simulink model "YMBOX_Control_Core"  (R2024b)
settings: Solver=FixedStepDiscrete  StartTime=0.0  StopTime=3  RelTol=1e-3
PreLoadFcn:
  | run(fullfile(fileparts(get_param(bdroot,'FileName')), 'YMBOX_Deluxe_init.m'));
InitFcn:
  | YMBOX_InitializeModel('core',bdroot);
model workspace (MAT data in the model file):
  KuMDAS_ObserverBuildVariant = Simulink.Parameter
  KuMDAS_ObserverBuildVariant.Value = 1
  KuMDAS_ObserverBuildVariant.Complexity = 'real'
  KuMDAS_ObserverBuildVariant.Dimensions = [1 1]
  KuMDAS_ObserverBuildVariant.Description = 'Product observer build Variant: 0=sensored-only, 1=SMO sensorless'
  KuMDAS_ObserverBuildVariant.DataType = 'uint8'
undefined symbols (not defined in the file or in its folder): CeMDSM_DrvModeIfStart_enum, CeMDSM_DrvModeSpdSens_enum, CeMDSM_DrvModeSpdSmo_enum, CeMDSM_DrvModeTrq_enum, Cf_CONTROL_TASK_TIME_S, KbMDAS_SmoDeadTimeCompEnable_flg, KbMDSA_ActiveInverterCompEnable_flg, KbMDSA_UnifiedVoltageLimitEnable_flg, KbMDSP_DCBusVoltReportFilterEnable_flg, KbMDTM_DAxisPriorityInFW_flg, KbMDTM_FieldWeakeningEnable_flg, KbMDTM_FinalIqAntiWindupEnable_flg, KbMDTM_SensorlessFieldWeakeningEnable_flg, KbMDTM_TorquePriorityBelowBase_flg, KbMDTM_UnifiedConstraintEnable_flg, KfMDAS_ControlCountToElecRad_NULL, KfMDAS_IfAccel_rpms, KfMDAS_IfAlignTime_s, KfMDAS_IfBlendTime_s, KfMDAS_IfSwitchSpd_rpm, KfMDAS_NativeCountToMechRad_NULL, KfMDAS_ObserverExitRatio_NULL, KfMDAS_SlsCtrlPeriod_s, KfMDAS_SlsEAngleInit_rad, KfMDAS_SlsElecSpdMax_rads, KfMDAS_SlsElecSpdMin_rads, KfMDAS_SlsTwoPi_rad, KfMDAS_SmoAngleOffset_rad, KfMDAS_SmoCurrentZohCoefA_NULL, KfMDAS_SmoCurrentZohCoefB_AperV, KfMDAS_SmoDeadTimeCurrentBoundary_A, KfMDAS_SmoDeadTimeDuty_NULL, KfMDAS_SmoDeadTimePolarity_NULL, KfMDAS_SmoDeviceDrop_V, KfMDAS_SmoEmfLpfCoefA_NULL, KfMDAS_SmoEmfLpfCoefB_NULL, KfMDAS_SmoEmfLpfInvPole_s, KfMDAS_SmoErrBoundaryMax_A, KfMDAS_SmoErrBoundarySpan_A, KfMDAS_SmoGainSchedAlpha_NULL, KfMDAS_SmoGainSchedAngleComp_rad, KfMDAS_SmoGainSchedEmfLow_V, KfMDAS_SmoGainSchedInvSpan_PerV, KfMDAS_SmoLdMinusLq_H, KfMDAS_SmoPllKiTs_NULL, KfMDAS_SmoPllKp_NULL, KfMDAS_SmoPllMinEmf_V, KfMDAS_SmoPllSpeedLpfAlpha_NULL, KfMDAS_SmoSlideGainMin_V, KfMDAS_SmoSlideGainSpan_V, KfMDAS_SmoSwitchSpd_rpm, KfMDAS_SmoTotalDelay_s, KfMDCC_DqSoftwareOverCurrentThreshold_A, KfMDCC_PiKcTsId_NULL, KfMDCC_PiKcTsIq_NULL, KfMDCC_PiKiTsId_NULL, KfMDCC_PiKiTsIq_NULL, KfMDCC_PiKpValueId_NULL, KfMDCC_PiKpValueIq_NULL, KfMDCC_PwmFreq_Hz ... (+84)
libraries: YMBOX_SharedMath_Lib x11, spsabctoAlphaBetaZeroLib x1
(part 1 of 8)
settings Model: Creator=ASUS  LastModifiedBy=ASUS
settings SolverCC: AlgebraicLoopSolver=TrustRegion  AutoInsertRateTranBlk=on
settings DataIOCC: LimitDataPoints=on  SaveFormat=StructureWithTime  SignalLoggingSaveFormat=ModelDataLogs  SaveOutput=off  SaveTime=off  ReturnWorkspaceOutputs=off
settings OptimizationCC: BlockReduction=off  ConditionallyExecuteInputs=off  DefaultParameterBehavior=Inlined  DefaultUnderspecifiedDataType=single  EnhancedBackFolding=on  PassReuseOutputArgsAs=Individual arguments  ExpressionDepthLimit=2147483647  InitFltsAndDblsToZero=on  EfficientFloat2IntCast=on  EfficientMapNaN2IntZero=off  OptimizeBlockOrder=speed  DifferentSizesBufferReuse=on  OptimizationCustomize=off  EfficientTunableParamExpr=on
settings DebuggingCC: ConsistencyChecking=warning  SignalInfNanChecking=error  SignalRangeChecking=error  SaveWithParameterizedLinksMsg=none  CheckSSInitialOutputMsg=off  UnderspecifiedInitializationDetection=Classic  MergeDetectMultiDrivingBlocksExec=none  TimeAdjustmentMsg=warning  MaxConsecutiveZCsMsg=warning  SolverPrmCheckMsg=warning  InheritedTsInSrcMsg=none  CheckMatrixSingularityMsg=error  ParameterOverflowMsg=warning  ParameterUnderflowMsg=error  ParameterPrecisionLossMsg=none  FixptConstUnderflowMsg=warning  FixptConstOverflowMsg=warning  FixptConstPrecisionLossMsg=warning  VectorMatrixConversionMsg=warning  FcnCallInpInsideContextMsg=warning  UnconnectedInputMsg=warning  UnconnectedOutputMsg=warning  UnconnectedLineMsg=warning  UniqueDataStoreMsg=warning  AllowSymbolicDim=off  StateNameClashWarn=warning  SFUnexpectedBacktrackingDiag=warning  SFNoUnconditionalDefaultTransitionDiag=warning  SFExecutionAtInitializationDiag=none  ArithmeticOperatorsInVariantConditions=warning
settings HardwareCC: ProdBitPerChar=16  ProdBitPerInt=16  ProdBitPerPointer=32  ProdBitPerSizeT=32  ProdBitPerPtrDiffT=32  ProdLargestAtomicInteger=Integer  ProdLargestAtomicFloat=None  ProdWordSize=16  ProdHWDeviceType=Texas Instruments->C2000  TargetIntDivRoundTo=Zero  TargetEndianess=LittleEndian  TargetHWDeviceType=Infineon->TriCore  ProdEqTarget=off
settings ModelReferenceCC: EnableRefExpFcnMdlSchedulingChecks=on  ModelReferenceNumInstancesAllowed=Single  PropagateSignalLabelsOutOfModel=off
settings SFSimCC: SimUseLocalCustomCode=off  MATLABDynamicMemAlloc=off  CustomCodeUndefinedFunction=UseInterfaceOnly
settings SFSimCC: SimCustomSourceCode=|
  | void Pwm_SetOutputToIdle_Now(void){};
  | void InverterDisable(void){};
  | void Pwm_Write(void){};
  | void InverterEnable(void){};
  | void vPwm_MDCC_UdUqCalc1_PI_Self_initialize(void){};
  | void SpeedLoopMode_initialize(void){};
settings SFSimCC: SimCustomHeaderCode=|
  | void Pwm_SetOutputToIdle_Now(void);
  | void InverterDisable(void);
  | void Pwm_Write(void);
  | void InverterEnable(void);
  | void vPwm_MDCC_UdUqCalc1_PI_Self_initialize(void);
  | void SpeedLoopMode_initialize(void);
  | #include "mdsa_sincos_f32.h"
  | #include "ymbox_atan_f32.h"
  | #include "ymbox_sqrt_f32.h"
  | #include "ymbox_scalar_math_f32.h"
settings SFSimCC: SimCustomInitializer=|
  | MDSA_SinCos_Init();
  | YMBOX_Atan_Init();
  | YMBOX_Sqrt_Init();
settings SFSimCC: SimUserSources=|
  | Platform/SinCos/mdsa_sincos_generic.c
  | Platform/Atan/ymbox_atan_generic.c
  | Platform/Sqrt/ymbox_sqrt_generic.c
  | Platform/SharedMath/ymbox_scalar_math_f32.c
settings SFSimCC: SimUserIncludeDirs=|
  | Platform/SinCos
  | Platform/Atan
  | Platform/Sqrt
  | Platform/SharedMath
settings RTWCC: Description=Embedded Coder  SystemTargetFile=ert.tlc  TLCOptions=-p0  GenCodeOnly=on  TemplateMakefile=ert_default_tmf  GenerateReport=on  RTWUseLocalCustomCode=off  IncludeHyperlinkInReport=on  GPUComputeCapability=3.5
settings RTWCC: CustomHeaderCode=|
  | extern void Pwm_SetOutputToIdle_Now(void);
  | extern void InverterDisable(void);
  | extern void Pwm_Write(void);
  | extern void InverterEnable(void);
  | void vPwm_MDCC_UdUqCalc1_PI_Self_initialize(void);
  | void SpeedLoopMode_initialize(void);
  | #include "mdsa_sincos_f32.h"
  | #include "ymbox_atan_f32.h"
  | #include "ymbox_sqrt_f32.h"
  | #include "ymbox_scalar_math_f32.h"
settings RTWCC: CustomInclude=|
  | Platform/SinCos
  | Platform/Atan
  | Platform/Sqrt
  | Platform/SharedMath
settings CodeAppCC: GenerateComments=off  IgnoreCustomStorageClasses=off  MaxIdLength=100  OperatorAnnotations=on  SFDataObjDesc=on  CustomSymbolStrGlobalVar=rt$N$M  CustomSymbolStrType=$N$M  CustomSymbolStrFcn=$N$M$F  CustomSymbolStrMacro=$N$M  CustomCommentsFcn=comments_mptfun.m  DefineNamingRule=UpperCase  SimulinkBlockComments=off  InternalIdentifier=Classic
settings ERTTargetCC: TargetLangStandard=C99 (ISO)  CodeReplacementLibrary=YMBOX single math  GenerateSampleERTMain=on  ERTCustomFileTemplate=example_file_process.tlc
settings ConfigComp: CovMetricSettings=dw  CovSaveCumulativeToWorkspaceVar=on  CovSaveSingleToWorkspaceVar=on  CovExternalEMLEnable=off

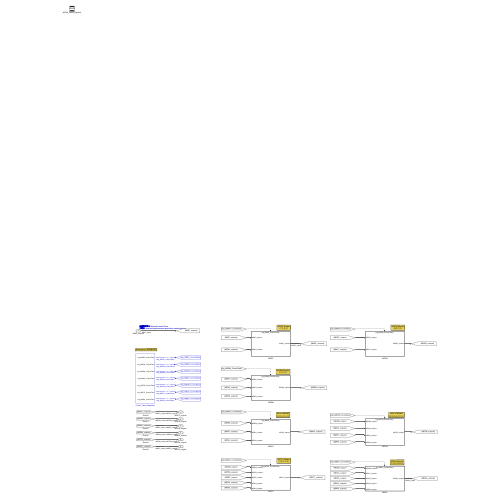
[thumbnail: Simulink's stored preview of the top-level diagram]
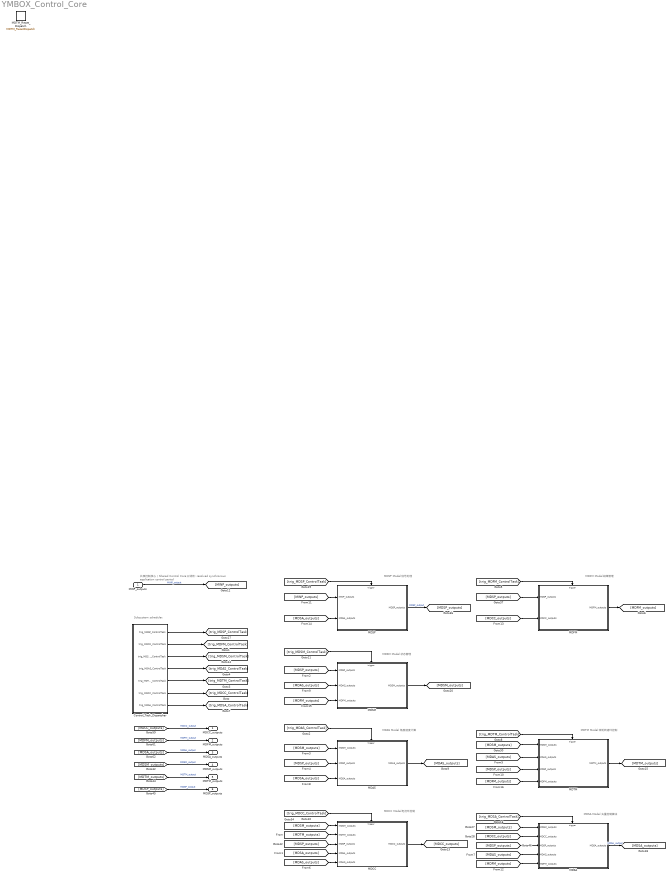
== system YMBOX_Control_Core ==
  note: Subsystem scheduler.
  note: MDFM Model
      | 故障管理
  note: MDCC Model
      | 电流环控制
  note: MDSA Model
      | 矢量控制算法
  note: MDTM Model
      | 转矩转速环控制
  note: MDSM Model
      | 状态管理
  note: MDAS Model
      | 角度速度计算
  note: 共享控制核心 / Shared Control Core
      | 父调用: resolved synchronous application control period
  note: MDSP Model
      | 信号处理
  MINP_outputs : Inport  OutDataTypeStr=Bus: MINP_output
  Control_Task_Dispatcher : Subsystem
  MDAS : Subsystem  TreatAsAtomicUnit=on  RTWFileName=AUXV_control
      settings: RTWSystemCode=Nonreusable function  RTWFileNameOpts=Use subsystem name
  MDCC : Subsystem  TreatAsAtomicUnit=on  RTWFileName=AUXV_control
      settings: RTWSystemCode=Nonreusable function  RTWFileNameOpts=Use subsystem name
  MDFM : Subsystem  TreatAsAtomicUnit=on  RTWFileName=AUXV_control
      settings: RTWSystemCode=Nonreusable function  RTWFileNameOpts=Use subsystem name
  MDSA : Subsystem  TreatAsAtomicUnit=on  RTWFileName=AUXV_control
      settings: RTWSystemCode=Nonreusable function  RTWFileNameOpts=Use subsystem name
  MDSM : Subsystem  TreatAsAtomicUnit=on  RTWFileName=AUXV_control
      settings: RTWSystemCode=Nonreusable function  RTWFileNameOpts=Use subsystem name
  MDSP : Subsystem
  MDTM : Subsystem  TreatAsAtomicUnit=on  RTWFileName=AUXV_control
      settings: RTWSystemCode=Nonreusable function  RTWFileNameOpts=Use subsystem name
  MDTM_Reset_Dispatch : DataStoreMemory  Description=MDSM writes the current fast-tick reset request before Scheduler reads it. Read only after trig_MDSM_ControlTask returns.  DataStoreName=MDTM_ResetDispatch  InitialValue=false  ShowAdditionalParam=off  OutDataTypeStr=boolean
  MDCC_outputs : Outport  OutDataTypeStr=Bus: MDCC_output
  MDFM_outputs : Outport  Port=2  OutDataTypeStr=Bus: MDFM_output
  MDSA_outputs : Outport  Port=3  OutDataTypeStr=Bus: MDSA_output
  MDSM_outputs : Outport  Port=4  OutDataTypeStr=Bus: MDSM_output
  MDTM_outputs : Outport  Port=5  OutDataTypeStr=Bus: MDTM_output
  MDSP_outputs : Outport  Port=6  OutDataTypeStr=Bus: MDSP_output
  wires:
  [MDFM_outputs] -> MDFM_outputs/1  "MDFM_output"
  [MDCC_outputs] -> MDCC_outputs/1  "MDCC_output"
  Control_Task_Dispatcher/5(trig_MDTM_ControlTask) -> [trig_MDTM_ControlTask]
  Control_Task_Dispatcher/7(trig_MDSA_ControlTask) -> [trig_MDSA_ControlTask]
  Control_Task_Dispatcher/6(trig_MDCC_ControlTask) -> [trig_MDCC_ControlTask]
  Control_Task_Dispatcher/2(trig_MDFM_ControlTask) -> [trig_MDFM_ControlTask]
  [MDSA_outputs] -> MDSA_outputs/1  "MDSA_output"
  Control_Task_Dispatcher/3(trig_MDSM_ControlTask) -> [trig_MDSM_ControlTask]
  [MDTM_outputs] -> MDTM_outputs/1  "MDTM_output"
  [MDSM_outputs] -> MDSM_outputs/1  "MDSM_output"
  [trig_MDFM_ControlTask] -> MDFM/Trigger
  MDFM/1(MDFM_outputs) -> [MDFM_outputs]
  [trig_MDCC_ControlTask] -> MDCC/Trigger
  MDCC/1(MDCC_outputs) -> [MDCC_outputs]
  [trig_MDSA_ControlTask] -> MDSA/Trigger
  MDSA/1(MDSA_outputs) -> [MDSA_outputs]  "MDSA_output"
  [trig_MDTM_ControlTask] -> MDTM/Trigger
  MDTM/1(MDTM_outputs) -> [MDTM_outputs]
  [trig_MDSM_ControlTask] -> MDSM/Trigger
  MDSM/1(MDSM_outputs) -> [MDSM_outputs]
  [MDSM_outputs] -> MDSA/1(MDSM_outputs)
  [MDCC_outputs] -> MDSA/2(MDCC_outputs)
  [MDSM_outputs] -> MDTM/1(MDSM_outputs)
  [MDSM_outputs] -> MDCC/1(MDSM_outputs)
  [MDTM_outputs] -> MDCC/2(MDTM_outputs)
  [MDSP_outputs] -> MDFM/1(MDSP_outputs)
  [MDSP_outputs] -> MDCC/3(MDSP_outputs)
  [MDSP_outputs] -> MDSA/3(MDSP_outputs)
  [MDSP_outputs] -> MDSP_outputs/1  "MDSP_output"
  [MDSP_outputs] -> MDSM/1(MDSP_outputs)
  [MDSA_outputs] -> MDCC/4(MDSA_outputs)
  Control_Task_Dispatcher/4(trig_MDAS_ControlTask) -> [trig_MDAS_ControlTask]
  [trig_MDAS_ControlTask] -> MDAS/Trigger
  [MDSM_outputs] -> MDAS/1(MDSM_outputs)
  [MDSP_outputs] -> MDAS/2(MDSP_outputs)
  MDAS/1(MDAS_outputs) -> [MDAS_outputs]
  [MDAS_outputs] -> MDTM/2(MDAS_outputs)
  [MDAS_outputs] -> MDCC/5(MDAS_outputs)
  [MDAS_outputs] -> MDSA/4(MDAS_outputs)
  [MDSA_outputs] -> MDAS/3(MDSA_outputs)
  [MDAS_outputs] -> MDSM/2(MDAS_outputs)
  [MDSP_outputs] -> MDTM/3(MDSP_outputs)
  MDSP/1(MDSP_outputs) -> [MDSP_outputs]  "MDSP_output"
  MINP_outputs/1 -> [MINP_outputs]  "MINP_output"
  [MINP_outputs] -> MDSP/1(MINP_outputs)
  [trig_MDSP_ControlTask] -> MDSP/Trigger
  Control_Task_Dispatcher/1(trig_MDSP_ControlTask) -> [trig_MDSP_ControlTask]
  [MDSA_outputs] -> MDSP/2(MDSA_outputs)
  [MDFM_outputs] -> MDSM/3(MDFM_outputs)
  [MDFM_outputs] -> MDTM/4(MDFM_outputs)
  [MDFM_outputs] -> MDSA/5(MDFM_outputs)
  [MDCC_outputs] -> MDFM/2(MDCC_outputs)

== system YMBOX_Control_Core/Control_Task_Dispatcher ==
  note: Scheduler to trigger the main application
      | sub-systems.
  Scheduler : Stateflow chart  TreatAsAtomicUnit=on
      settings: PortSchema="{\"entries\":[{\"content\":{\"sides\":[{\"content\":{},\"type\":\"ConnectorPlacement.EquallySpacedRectSide\",\"uuid\":\"ed742335-5841-4393-a6a4-c33eaa575858\"},{\"content\":{\"connectorIds\":[\"Out7\",\"Out1\",\"Out2\",\"Out3\",\"Out4\",\"Out5\",\"Out6\"],\"side\":\"RIGHT\"},\"type\":\"ConnectorPlacement.EquallySpacedRectSide\",\"uuid\":\"a5f78643-cf3a-43ed-917c-1379891acf9e\"},{\"content\":{\"side\":\"TOP\"},\"type\":\"ConnectorPlacement.EquallySpacedRectSide\",\"uuid\":\"5ceff9a0-c2d2-40e1-aa51-0f4c65c30636\"}]},\"type\":\"ConnectorPlacement.EquallySpacedConnector\",\"uuid\":\"5d18fd33-d652-411a-b3bb-ce8a67e81c97\"}],\"packageUris\":[\"http://schema.mathworks.com/mf0/Connector/R2020b\"],\"version\":\"1.0\"}"
  trig_MDSP_ControlTask : Outport
  trig_MDFM_ControlTask : Outport  Port=2
  trig_MDSM_ControlTask : Outport  Port=3
  trig_MDAS_ControlTask : Outport  Port=4
  trig_MDTM_ControlTask : Outport  Port=5
  trig_MDCC_ControlTask : Outport  Port=6
  trig_MDSA_ControlTask : Outport  Port=7
  wires:
  Scheduler/1(trig_MDFM_ControlTask()) -> trig_MDFM_ControlTask/1
  Scheduler/2(trig_MDSM_ControlTask()) -> trig_MDSM_ControlTask/1
  Scheduler/3(trig_MDAS_ControlTask()) -> trig_MDAS_ControlTask/1
  Scheduler/4(trig_MDTM_ControlTask()) -> trig_MDTM_ControlTask/1
  Scheduler/5(trig_MDCC_ControlTask()) -> trig_MDCC_ControlTask/1
  Scheduler/6(trig_MDSA_ControlTask()) -> trig_MDSA_ControlTask/1
  Scheduler/7(trig_MDSP_ControlTask()) -> trig_MDSP_ControlTask/1

== system YMBOX_Control_Core/MDAS ==
  MDSM_outputs : Inport
  MDSP_outputs : Inport  Port=2
  MDSA_outputs : Inport  Port=3
  trig_MDAS_ControlTask : TriggerPort  TriggerType=function-call  VariantControl=(inherit)
  Bus Creator : BusCreator  Inputs=12  OutDataTypeStr=Bus: MDAS_output
  Bus Selector : BusSelector  OutputSignals=VeMDSM_DrvModeCmd_enum,VeMDSM_DrvModeReq_enum,VfMDSM_TrgtSpd_rpm
  Bus Selector1 : BusSelector  OutputSignals=Resolver_Output.VuMDSP_MotMechAngleRaw_NULL
  IF_Startup_Internal : Subsystem  Variant=on
      settings: AttributesFormatString=PRODUCT BUILD VARIANT\n0 SENSORED | 1 SMO
  MDAS_DriveModeRoute_Variant : Subsystem  Variant=on
      settings: AttributesFormatString=PRODUCT BUILD VARIANT\n0 SENSORED | 1 SMO
  MechSpd_To_ElecSpd : Gain  Gain=single(KuMDMP_Pole_Pair_Number_NULL)  OutDataTypeStr=single
  Position_Feedback_Status : Stateflow chart  TreatAsAtomicUnit=on
  Position_NativeCountToMechRad : Constant  Value=KfMDAS_NativeCountToMechRad_NULL
  Position_TwoPiRad : Constant  Value=KfMDAS_SlsTwoPi_rad
  Sensorless_FluxMRAS : Subsystem  Variant=on  VariantControl=Sensorless_FluxMRAS
      settings: AttributesFormatString=PRODUCT BUILD VARIANT\n0 SENSORED | 1 SMO
  MDAS_outputs : Outport  OutDataTypeStr=Bus: MDAS_output
  wires:
  MDSM_outputs/1 -> Bus Selector/1, Sensorless_FluxMRAS/3(MDSM_outputs)
  [MDAS_SMO_ELEC_ANGLE_RAD_ROUTE] -> MDAS_DriveModeRoute_Variant/8(VfMDAS_SmoAlignedElecAngle_rad)
  MDSA_outputs/1 -> Sensorless_FluxMRAS/2(MDSA_outputs)
  [MDAS_RAW_ANGLE_ROUTE] -> Position_Feedback_Status/2(rawMechCount), MDAS_DriveModeRoute_Variant/2(<VuMDSP_MotMechAngleRaw_NULL>)
  [MDAS_SMO_ABS_ROUTE] -> MDAS_DriveModeRoute_Variant/5(VfMDAS_SmoMechSpdAbs_rads)
  MDSP_outputs/1 -> Bus Selector1/1, Sensorless_FluxMRAS/1(MDSP_outputs)
  [MDAS_IF_ABS_ROUTE] -> MDAS_DriveModeRoute_Variant/3(VfMDAS_IfMechSpdAbs_rads)
  [MDAS_MODE_CMD_ROUTE] -> MDAS_DriveModeRoute_Variant/1(<VeMDSM_DrvModeCmd_enum>), Position_Feedback_Status/1(modeCmd)
  [MDAS_IF_ELEC_ANGLE_RAD_ROUTE] -> MDAS_DriveModeRoute_Variant/7(VfMDAS_IfElecAngle_rad)
  [MDAS_IF_SPD_ROUTE] -> MDAS_DriveModeRoute_Variant/4(VfMDAS_IfMechSpd_rads)
  [MDAS_READY_BUS] -> Bus Creator/4, Position_Feedback_Status/5(smoReady)
  [MDAS_SMO_SPD_ROUTE] -> MDAS_DriveModeRoute_Variant/6(VfMDAS_SmoMechSpd_rads)
  Bus Selector/1 -> [MDAS_MODE_CMD_ROUTE], IF_Startup_Internal/1(VeMDAS_DrvModeCmd_enum)  "<VeMDSM_DrvModeCmd_enum>"
  Position_Feedback_Status/1(mechAngleRad) -> Bus Creator/7  "VfMDAS_MotMechAngle_rad"
  Bus Selector/2 -> IF_Startup_Internal/2(VeMDAS_DrvModeReq_enum)  "<VeMDSM_DrvModeReq_enum>"
  Bus Selector1/1 -> [MDAS_RAW_ANGLE_ROUTE]  "<VuMDSP_MotMechAngleRaw_NULL>"
  Bus Selector/3 -> IF_Startup_Internal/3(VfMDAS_TargetSpd_rpm)  "<VfMDSM_TrgtSpd_rpm>"
  Sensorless_FluxMRAS/1(VfMDAS_SmoElecAngle_rad) -> IF_Startup_Internal/4(VfMDAS_SmoElecAngle_rad)
  Sensorless_FluxMRAS/2(VfMDAS_SmoElecSpd_rads) -> IF_Startup_Internal/5(VfMDAS_SmoElecSpd_rads)
  IF_Startup_Internal/9(VfMDAS_HandoverElecAngleDelta_rad) -> [MDAS_HANDOVER_ELEC_ANGLE_DELTA_RAD]  "VfMDAS_HandoverElecAngleDelta_rad"
  Sensorless_FluxMRAS/3(VfMDAS_SmoEmfMag_V) -> IF_Startup_Internal/6(VfMDAS_SmoEmfMag_V)
  IF_Startup_Internal/4(VfMDAS_SmoMechSpd_rads) -> [MDAS_SMO_SPD_ROUTE]  "VfMDAS_SmoMechSpd_rads"
  IF_Startup_Internal/3(VfMDAS_IfElecAngle_rad) -> [MDAS_IF_ELEC_ANGLE_RAD_ROUTE]  "VfMDAS_IfElecAngle_rad"
  IF_Startup_Internal/2(VfMDAS_IfMechSpdAbs_rads) -> [MDAS_IF_ABS_ROUTE]  "VfMDAS_IfMechSpdAbs_rads"
  IF_Startup_Internal/1(VfMDAS_IfMechSpd_rads) -> [MDAS_IF_SPD_ROUTE]  "VfMDAS_IfMechSpd_rads"
  Sensorless_FluxMRAS/4(VfMDAS_SmoPllPhaseErr_NULL) -> IF_Startup_Internal/7(VfMDAS_SmoPllPhaseErr_NULL)
  MDAS_DriveModeRoute_Variant/3(VfMDAS_SelectedElecAngle_rad) -> Position_Feedback_Status/3(selectedElecAngleRad)  "VfMDAS_SelectedElecAngle_rad"
  MDAS_DriveModeRoute_Variant/2(VfMDAS_MotMechSpdFiltered_rads) -> Position_Feedback_Status/4(selectedMechSpdRads), Bus Creator/1, MechSpd_To_ElecSpd/1  "VfMDAS_MotMechSpdFiltered_rads"
  MDAS_DriveModeRoute_Variant/1(VfMDAS_MotMechSpdFilteredAbs_rads) -> Bus Creator/2  "VfMDAS_MotMechSpdFilteredAbs_rads"
  Position_NativeCountToMechRad/1 -> Position_Feedback_Status/6(nativeToMech)
  Position_TwoPiRad/1 -> Position_Feedback_Status/7(twoPiRad)
  IF_Startup_Internal/8(VfMDAS_HandoverBlend_NULL) -> [MDAS_BLEND_BUS]  "VfMDAS_HandoverBlend_NULL"
  IF_Startup_Internal/7(VfMDAS_SmoAlignedElecAngle_rad) -> [MDAS_SMO_ELEC_ANGLE_RAD_ROUTE]  "VfMDAS_SmoAlignedElecAngle_rad"
  IF_Startup_Internal/6(VbMDAS_SmoReady_flg) -> [MDAS_READY_BUS]  "VbMDAS_SmoReady_flg"
  IF_Startup_Internal/5(VfMDAS_SmoMechSpdAbs_rads) -> [MDAS_SMO_ABS_ROUTE]  "VfMDAS_SmoMechSpdAbs_rads"
  MechSpd_To_ElecSpd/1 -> Bus Creator/3  "VfMDAS_MotElecSpd_rads"
  [MDAS_BLEND_BUS] -> Bus Creator/5
  [MDAS_HANDOVER_ELEC_ANGLE_DELTA_RAD] -> Bus Creator/6
  Position_Feedback_Status/2(elecAngleRad) -> Bus Creator/8  "VfMDAS_MotElecAngle_rad"
  Position_Feedback_Status/3(angleValid) -> Bus Creator/9  "VbMDAS_PositionAngleValid_flg"
  Position_Feedback_Status/4(speedValid) -> Bus Creator/10  "VbMDAS_PositionSpeedValid_flg"
  Position_Feedback_Status/5(quality) -> Bus Creator/11  "VfMDAS_PositionQuality_NULL"
  Bus Creator/1 -> MDAS_outputs/1
  Position_Feedback_Status/6(direction) -> Bus Creator/12  "VeMDAS_PositionDirection_enum"

== system YMBOX_Control_Core/MDCC ==
  MDSM_outputs : Inport
  MDTM_outputs : Inport  Port=2
  MDSP_outputs : Inport  Port=3
  MDSA_outputs : Inport  Port=4
  MDAS_outputs : Inport  Port=5
  trig_MDCC_ControlTask : TriggerPort  TriggerType=function-call  VariantControl=(inherit)
  Bus Creator : BusCreator  Inputs=7
  Bus Selector1 : BusSelector  OutputSignals=VeMDSM_DrvModeCmd_enum
  Bus Selector2 : BusSelector  OutputSignals=VfMDTM_IdCmd_A,VfMDTM_IqCmd_A
  Bus Selector3 : BusSelector  OutputSignals=Direct_Output.VMIN_Dir_TestUaUdId_NULL,Direct_Output.VMIN_Dir_TestUbUqIq_NULL
  Bus Selector4 : BusSelector  OutputSignals=VfMDSP_PhaseUCurrentCtrl_A,VfMDSP_PhaseVCurrentCtrl_A,VfMDSP_PhaseWCurrentCtrl_A
  Bus Selector5 : BusSelector  OutputSignals=VfMDAS_MotElecAngle_rad
  Bus Selector7 : BusSelector  OutputSignals=VfMDAS_MotMechSpdFiltered_rads
  Bus Selector8 : BusSelector  OutputSignals=VbMDCC_PiReset_flg,VeMDFM_FFEnable_enum
  Bus Selector9 : BusSelector  OutputSignals=VfMDSA_k_effective_NULL
  MDCC_Subsystem : Subsystem  TreatAsAtomicUnit=on  RTWFcnName=vPwm_MDCC  RTWFileName=MDCC
      settings: RTWSystemCode=Nonreusable function  RTWFcnNameOpts=User specified  RTWFileNameOpts=User specified
  MDCC_outputs : Outport
  wires:
  MDAS_outputs/1 -> [MDAS_outputs]
  Bus Selector9/1 -> MDCC_Subsystem/13(VfMDCC_k_effective_NULL)  "<VfMDSA_k_effective_NULL>"
  [MDSA_outputs] -> Bus Selector9/1
  MDSA_outputs/1 -> [MDSA_outputs]
  Bus Selector2/2 -> MDCC_Subsystem/4(VfMDCC_QCurCmd_A)  "<VfMDTM_IqCmd_A>"
  Bus Selector2/1 -> MDCC_Subsystem/3(VfMDCC_DCurCmd_A)  "<VfMDTM_IdCmd_A>"
  MDCC_Subsystem/5(VfMDCC_QCur_A) -> Bus Creator/5
  MDCC_Subsystem/4(VfMDCC_DCur_A) -> Bus Creator/4
  MDCC_Subsystem/3(VbMDCC_DqSoftwareOverCurrent_flg) -> Bus Creator/3
  MDCC_Subsystem/2(VfMDCC_VoltQ_V) -> Bus Creator/2  "VfMDCC_VoltQ_V"
  MDCC_Subsystem/1(VfMDCC_VoltD_V) -> Bus Creator/1  "VfMDCC_VoltD_V"
  Bus Selector3/2 -> MDCC_Subsystem/10(VfMDCC_TestUbetaUqIq_NULL)  "<VMIN_Dir_TestUbUqIq_NULL>"
  Bus Selector7/1 -> MDCC_Subsystem/5(VfMDCC_MotMechSpdFiltered_rads)  "<VfMDAS_MotMechSpdFiltered_rads>"
  Bus Selector8/2 -> MDCC_Subsystem/12(VuMDCC_FFEnable_enum)  "<VeMDFM_FFEnable_enum>"
  Bus Selector8/1 -> MDCC_Subsystem/11(VbMDCC_PiReset_flg)  "<VbMDCC_PiReset_flg>"
  [MDSM_outputs] -> Bus Selector8/1
  Bus Selector3/1 -> MDCC_Subsystem/9(VfMDCC_TestUalphaUdId_NULL)  "<VMIN_Dir_TestUaUdId_NULL>"
  Bus Selector4/3 -> MDCC_Subsystem/8(VfMDCC_WCur_A)  "<VfMDSP_PhaseWCurrentCtrl_A>"
  Bus Selector4/2 -> MDCC_Subsystem/7(VfMDCC_VCur_A)  "<VfMDSP_PhaseVCurrentCtrl_A>"
  Bus Selector4/1 -> MDCC_Subsystem/6(VfMDCC_UCur_A)  "<VfMDSP_PhaseUCurrentCtrl_A>"
  [MDAS_outputs] -> Bus Selector7/1
  [MDAS_outputs] -> Bus Selector5/1
  [MDSP_outputs] -> Bus Selector4/1
  [MDSP_outputs] -> Bus Selector3/1
  MDSP_outputs/1 -> [MDSP_outputs]
  [MDTM_outputs] -> Bus Selector2/1
  [MDSM_outputs] -> Bus Selector1/1
  MDTM_outputs/1 -> [MDTM_outputs]
  MDSM_outputs/1 -> [MDSM_outputs]
  Bus Selector1/1 -> MDCC_Subsystem/1(VeMDCC_DrvModeCmd_enum)  "<VeMDSM_DrvModeCmd_enum>"
  Bus Selector5/1 -> MDCC_Subsystem/2(VfMDCC_MotElecAngle_rad)  "<VfMDAS_MotElecAngle_rad>"
  Bus Creator/1 -> MDCC_outputs/1  "MDCC_output"
  MDCC_Subsystem/6(VfMDCC_EAngleCos_NULL) -> Bus Creator/6  "VfMDCC_EAngleCos_NULL"
  MDCC_Subsystem/7(VfMDCC_EAngleSin_NULL) -> Bus Creator/7  "VfMDCC_EAngleSin_NULL"

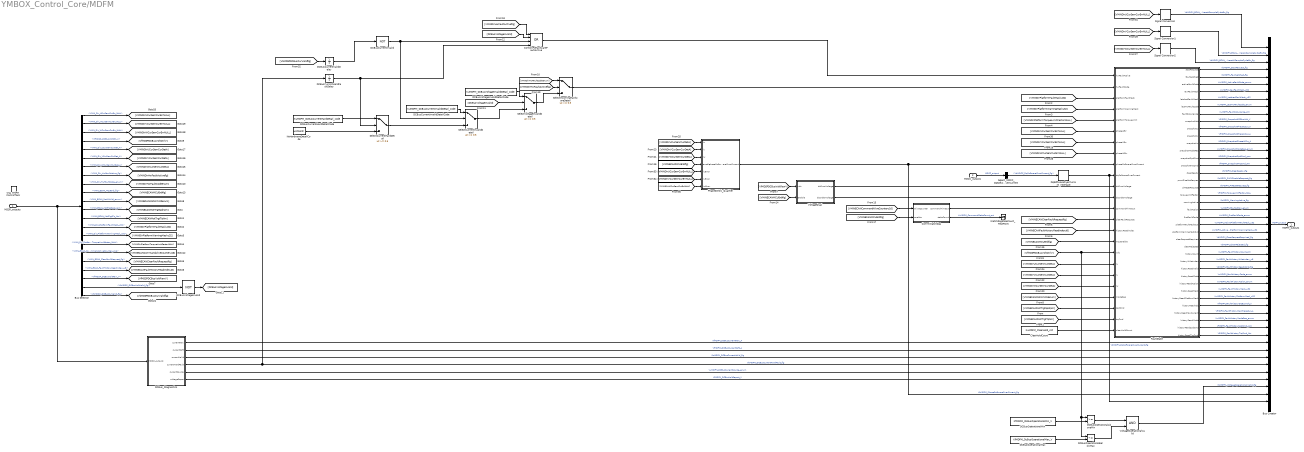
== system YMBOX_Control_Core/MDFM ==
  MDSP_outputs : Inport
  MDCC_outputs : Inport  Port=2  OutDataTypeStr=Bus: MDCC_output
  trig_MDFM_ControlTask : TriggerPort  TriggerType=function-call  VariantControl=(inherit)
  Bus Creator : BusCreator  Inputs=49
  Bus Selector : BusSelector  OutputSignals=Direct_Output.VMIN_Dir_UCurSenrCurErr_NULL,Direct_Output.VMIN_Dir_VCurSenrCurErr_NULL,Direct_Output.VMIN_Dir_WCurSenrCurErr_NULL,VfMDSP_DCBusVoltCtrl_V,Direct_Output.VMIN_Dir_UCurSenrCurDet_A,Direct_Output.VMIN_Dir_VCurSenrCurDet_A,Direct_Output.VMIN_Dir_WCurSenrCurDet_A,Direct_Output.VMIN_Dir_HwFaultActive_flg,Direct_Output.VMIN_Dir_HwFaultCode_enum,Direct_Output.VMIN_ECAN_MCUEnb_flg,Direct_Output.VMIN_ECAN_MotWrkMd_enum,Direct_Output.VMIN_ECAN_MotTrgtSpd_rpm,Direct_Output.VMIN_ECAN_MotTrgtTq_Nm,Direct_Output.VMIN_Dir_PlatformFaultMask_u32,Direct_Output.VMIN_Dir_PlatformWarningMask_u32,Direct_Output.VMIN_Dir_PlatformTorqueLimitFactor_NULL,Direct_Output.VMIN_ECAN_CommandAliveCounter_u16,Direct_Output.VMIN_ECAN_ClearFaultRequest_flg,Direct_Output.VMIN_ECAN_FaultHistoryReadIndex_u8,VfMDSP_DCBusVoltRaw_V,VbMDSP_DCBusVoltValid_flg,VbMDSP_DCBusCurValid_flg
  ClearHoldCount : Constant  Value=KuMDFM_ClearHold_cnt  OutDataTypeStr=uint32
  CombinedHardwareFaultActive : Logic  Operator=OR  Inputs=4
  CommWatchdog : Subsystem
  DCBusCurrentHardDetailCode : Constant  Value=KuMDFM_DcBusCurrentHardDetail_code
  DCBusCurrentHardFaultDelay : UnitDelay  InitialCondition=false  SampleTime=-1
  DCBusCurrentInvalid : Logic  Operator=NOT  Inputs=1
  DCBusCurrentInvalidDetailCode : Constant  Value=KuMDFM_DcBusCurrentInvalidDetail_code
  DCBusCurrentValidDelay : UnitDelay  InitialCondition=true  SampleTime=-1
  DCBusOperationalAboveMin : RelationalOperator
  DCBusOperationalBelowMax : RelationalOperator  Operator=<=
  DCBusOperationalMax : Constant  Value=KfMDFM_DcBusOperationalMax_V  OutDataTypeStr=single
  DCBusOperationalMin : Constant  Value=KfMDFM_DcBusOperationalMin_V  OutDataTypeStr=single
  DCBusVoltageInvalid : Logic  Operator=NOT  Inputs=1
  DCBusVoltageInvalidDetailCode : Constant  Value=KuMDFM_DcBusVoltageInvalidDetail_code
  DCBus_Diagnostics : Subsystem
  DqSoftwareOverCurrent_Interface : SignalConversion  OverrideOpt=off
  FaultState : MATLAB Function  TreatAsAtomicUnit=on
  NoHardwareDetailCode : Constant  Value=uint16(0)
  PhaseSWOC_Qualifier : Subsystem
  SelectCurrentHardDetail : Switch  Threshold=0.5
  SelectCurrentInvalidDetail : Switch  Threshold=0.5
  SelectIncomingHardwareDetail : Switch  Threshold=0.5
  SelectVoltageInvalidDetail : Switch  Threshold=0.5
  Select_MDCC_DqSoftwareOverCurrent : BusSelector  OutputSignals=VbMDCC_DqSoftwareOverCurrent_flg
  Signal Conversion : SignalConversion  OverrideOpt=off
  Signal Conversion1 : SignalConversion  OverrideOpt=off
  Signal Conversion2 : SignalConversion  OverrideOpt=off
  VoltageOperationalValid : Logic
  VoltageQual : Subsystem
  WatchdogStaleCount_TestPoint : Terminator
  MDFM_outputs : Outport
  wires:
  NoHardwareDetailCode/1 -> SelectCurrentHardDetail/3
  DCBusCurrentHardDetailCode/1 -> SelectCurrentHardDetail/1
  FaultState/29(historyReadCode) -> Bus Creator/32  "VuMDFM_FaultHistoryCode_enum"
  DCBusCurrentHardFaultDelay/1 -> CombinedHardwareFaultActive/4, SelectCurrentHardDetail/2
  SelectCurrentInvalidDetail/1 -> SelectVoltageInvalidDetail/3
  Signal Conversion1/1 -> Bus Creator/2  "VbMDFM_ECAN_PhaseVSampleCycleErr_flg"
  DCBusCurrentValidDelay/1 -> DCBusCurrentInvalid/1
  SelectVoltageInvalidDetail/1 -> SelectIncomingHardwareDetail/3
  MDSP_outputs/1 -> Bus Selector/1, DCBus_Diagnostics/1(MDSP_outputs)
  DCBusCurrentInvalid/1 -> SelectCurrentInvalidDetail/2, CombinedHardwareFaultActive/3
  DCBusCurrentInvalidDetailCode/1 -> SelectCurrentInvalidDetail/1
  FaultState/9(snapshotIu) -> Bus Creator/12  "VfMDFM_SnapshotPhaseUCur_A"
  Bus Selector/21 -> DCBusVoltageInvalid/1  "<VbMDSP_DCBusVoltValid_flg>"
  SelectCurrentHardDetail/1 -> SelectCurrentInvalidDetail/3
  VoltageQual/2(dcUnderVoltage) -> FaultState/12(dcUnderVoltage)
  FaultState/1(stopRequest) -> Bus Creator/4  "VbMDFM_StopRequest_flg"
  FaultState/16(pwmDisableRequest) -> Bus Creator/19  "VbMDFM_PWMDisableRequest_flg"
  SelectIncomingHardwareDetail/1 -> FaultState/2(hwFaultCode)
  FaultState/7(faultOccurrence) -> Bus Creator/10  "VuMDFM_FaultOccurrence_cnt"
  DCBusVoltageInvalidDetailCode/1 -> SelectVoltageInvalidDetail/1
  FaultState/11(snapshotIw) -> Bus Creator/14  "VfMDFM_SnapshotPhaseWCur_A"
  PhaseSWOC_Qualifier/1(phaseSoftwareOverCurrent) -> Bus Creator/48, FaultState/9(phaseSoftwareOverCurrent)  "VbMDFM_PhaseSoftwareOverCurrent_flg"
  VoltageQual/1(dcOverVoltage) -> FaultState/11(dcOverVoltage)
  FaultState/5(latchedFaultMask) -> Bus Creator/8  "VuMDFM_LatchedFaultMask_u32"
  CommWatchdog/1(commandTimeout) -> FaultState/13(commandTimeout)
  CommWatchdog/2(staleCount) -> WatchdogStaleCount_TestPoint/1  "VuMDFM_CommandStaleCount_cnt"
  FaultState/15(clearReady) -> Bus Creator/18  "VbMDFM_ClearReady_flg"
  CombinedHardwareFaultActive/1 -> FaultState/1(hwFaultActive)
  ClearHoldCount/1 -> FaultState/24(clearHoldCount)
  FaultState/12(snapshotModeReq) -> Bus Creator/15  "VuMDFM_SnapshotModeReq_enum"
  Signal Conversion/1 -> Bus Creator/1  "VbMDFM_ECAN_PhaseUSampleCycleErr_flg"
  Signal Conversion2/1 -> Bus Creator/3  "VbMDFM_ECAN_PhaseWSampleCycleErr_flg"
  FaultState/13(snapshotSpdCmd) -> Bus Creator/16  "VfMDFM_SnapshotSpdCmd_rpm"
  FaultState/2(faultLatched) -> Bus Creator/5  "VbMDFM_FaultLatched_flg"
  FaultState/3(activeFaultCode) -> Bus Creator/6  "VuMDFM_ActiveFaultCode_enum"
  FaultState/4(rawFaultMask) -> Bus Creator/7  "VuMDFM_RawFaultMask_u32"
  FaultState/6(lastHwFaultCode) -> Bus Creator/9  "VuMDFM_LastHwFaultCode_enum"
  FaultState/8(snapshotVdc) -> Bus Creator/11  "VfMDFM_SnapshotDCBusVolt_V"
  FaultState/10(snapshotIv) -> Bus Creator/13  "VfMDFM_SnapshotPhaseVCur_A"
  FaultState/14(snapshotTrqCmd) -> Bus Creator/17  "VfMDFM_SnapshotTrqCmd_Nm"
  FaultState/17(piResetRequest) -> Bus Creator/20  "VbMDFM_PIResetRequest_flg"
  FaultState/18(torqueLimitFactor) -> Bus Creator/21  "VfMDFM_TorqueLimitFactor_NULL"
  FaultState/19(warningActive) -> Bus Creator/22  "VbMDFM_WarningActive_flg"
  FaultState/20(faultAction) -> Bus Creator/23  "VuMDFM_FaultAction_enum"
  FaultState/21(firstFaultCode) -> Bus Creator/24  "VuMDFM_FirstFaultCode_enum"
  FaultState/22(platformFaultMaskOut) -> Bus Creator/25  "VuMDFM_ActivePlatformFaultMask_u32"
  FaultState/23(platformWarningMaskOut) -> Bus Creator/26  "VuMDFM_ActivePlatformWarningMask_u32"
  FaultState/24(clearRequestRequired) -> Bus Creator/27  "VbMDFM_ClearRequestRequired_flg"
  FaultState/25(clearRejected) -> Bus Creator/28  "VbMDFM_ClearRejected_flg"
  FaultState/26(historyCount) -> Bus Creator/29  "VuMDFM_FaultHistoryCount_cnt"
  FaultState/27(historyWriteIndex) -> Bus Creator/30  "VuMDFM_FaultHistoryWriteIndex_u8"
  FaultState/28(historyReadValid) -> Bus Creator/31  "VbMDFM_FaultHistoryReadValid_flg"
  FaultState/30(historyReadAction) -> Bus Creator/33  "VuMDFM_FaultHistoryAction_enum"
  FaultState/31(historyReadMask) -> Bus Creator/34  "VuMDFM_FaultHistoryMask_u32"
  FaultState/32(historyReadPlatformMask) -> Bus Creator/35  "VuMDFM_FaultHistoryPlatformMask_u32"
  FaultState/33(historyReadVdc) -> Bus Creator/36  "VfMDFM_FaultHistoryDCBusVolt_V"
  FaultState/34(historyReadMaxCurrent) -> Bus Creator/37  "VfMDFM_FaultHistoryMaxPhaseCur_A"
  FaultState/35(historyReadMode) -> Bus Creator/38  "VuMDFM_FaultHistoryModeReq_enum"
  FaultState/36(historyReadSpdCmd) -> Bus Creator/39  "VfMDFM_FaultHistorySpdCmd_rpm"
  FaultState/37(historyReadTrqCmd) -> Bus Creator/40  "VfMDFM_FaultHistoryTrqCmd_Nm"
  Bus Creator/1 -> MDFM_outputs/1  "MDFM_output"
  Bus Selector/12 -> [VMINECANMotTrgtSpdrpm]  "<VMIN_ECAN_MotTrgtSpd_rpm>"
  [VMINECANMotTrgtSpdrpm] -> FaultState/22(spdCmd)
  Bus Selector/13 -> [VMINECANMotTrgtTqNm]  "<VMIN_ECAN_MotTrgtTq_Nm>"
  [VMINECANMotTrgtTqNm] -> FaultState/23(trqCmd)
  Bus Selector/14 -> [VMINDirPlatformFaultMasku32]  "<VMIN_Dir_PlatformFaultMask_u32>"
  [VMINDirPlatformFaultMasku32] -> FaultState/3(platformFaultMask)
  Bus Selector/15 -> [VMINDirPlatformWarningMasku32]  "<VMIN_Dir_PlatformWarningMask_u32>"
  [VMINDirPlatformWarningMasku32] -> FaultState/4(platformWarningMask)
  Bus Selector/16 -> [VMINDirPlatformTorqueLimitFactorNULL]  "<VMIN_Dir_PlatformTorqueLimitFactor_NULL>"
  [VMINDirPlatformTorqueLimitFactorNULL] -> FaultState/5(platformTorqueLimit)
  Bus Selector/18 -> [VMINECANClearFaultRequestflg]  "<VMIN_ECAN_ClearFaultRequest_flg>"
  [VMINECANClearFaultRequestflg] -> FaultState/14(clearFaultRequest)
  Bus Selector/19 -> [VMINECANFaultHistoryReadIndexu8]  "<VMIN_ECAN_FaultHistoryReadIndex_u8>"
  [VMINECANFaultHistoryReadIndexu8] -> FaultState/15(historyReadIndex)
  Bus Selector/20 -> [VfMDSPDCBusVoltRawV]  "<VfMDSP_DCBusVoltRaw_V>"
  [VfMDSPDCBusVoltRawV] -> VoltageQual/1(vdc)
  Bus Selector/11 -> [VMINECANMotWrkMdenum]  "<VMIN_ECAN_MotWrkMd_enum>"
  [VMINECANMotWrkMdenum] -> FaultState/21(modeReq)
  Bus Selector/4 -> [VfMDSPDCBusVoltCtrlV]  "<VfMDSP_DCBusVoltCtrl_V>"
  [VfMDSPDCBusVoltCtrlV] -> FaultState/17(vdc), DCBusOperationalBelowMax/1, DCBusOperationalAboveMin/1
  Bus Selector/9 -> [VMINDirHwFaultCodeenum]  "<VMIN_Dir_HwFaultCode_enum>"
  [VMINDirHwFaultCodeenum] -> SelectIncomingHardwareDetail/1
  DCBusVoltageInvalid/1 -> [DCBusVoltageInvalid]
  [DCBusVoltageInvalid] -> SelectVoltageInvalidDetail/2
  [DCBusVoltageInvalid] -> CombinedHardwareFaultActive/2
  Bus Selector/17 -> [VMINECANCommandAliveCounteru16]  "<VMIN_ECAN_CommandAliveCounter_u16>"
  [VMINECANCommandAliveCounteru16] -> CommWatchdog/1(aliveCounter)
  Bus Selector/10 -> [VMINECANMCUEnbflg]  "<VMIN_ECAN_MCUEnb_flg>"
  [VMINECANMCUEnbflg] -> VoltageQual/2(enable)
  [VMINECANMCUEnbflg] -> FaultState/16(mcuEnable)
  [VMINECANMCUEnbflg] -> PhaseSWOC_Qualifier/4(enable)
  [VMINECANMCUEnbflg] -> CommWatchdog/2(enable)
  Bus Selector/8 -> [VMINDirHwFaultActiveflg]  "<VMIN_Dir_HwFaultActive_flg>"
  [VMINDirHwFaultActiveflg] -> CombinedHardwareFaultActive/1
  [VMINDirHwFaultActiveflg] -> SelectIncomingHardwareDetail/2
  Bus Selector/7 -> [VMINDirWCurSenrCurDetA]  "<VMIN_Dir_WCurSenrCurDet_A>"
  [VMINDirWCurSenrCurDetA] -> FaultState/20(iw)
  [VMINDirWCurSenrCurDetA] -> PhaseSWOC_Qualifier/3(iw)
  Bus Selector/6 -> [VMINDirVCurSenrCurDetA]  "<VMIN_Dir_VCurSenrCurDet_A>"
  [VMINDirVCurSenrCurDetA] -> FaultState/19(iv)
  [VMINDirVCurSenrCurDetA] -> PhaseSWOC_Qualifier/2(iv)
  Bus Selector/5 -> [VMINDirUCurSenrCurDetA]  "<VMIN_Dir_UCurSenrCurDet_A>"
  [VMINDirUCurSenrCurDetA] -> FaultState/18(iu)
  [VMINDirUCurSenrCurDetA] -> PhaseSWOC_Qualifier/1(iu)
  Bus Selector/3 -> [VMINDirWCurSenrCurErrNULL]  "<VMIN_Dir_WCurSenrCurErr_NULL>"
  [VMINDirWCurSenrCurErrNULL] -> FaultState/8(phaseWErr)
  [VMINDirWCurSenrCurErrNULL] -> Signal Conversion2/1
  Bus Selector/2 -> [VMINDirVCurSenrCurErrNULL]  "<VMIN_Dir_VCurSenrCurErr_NULL>"
  [VMINDirVCurSenrCurErrNULL] -> FaultState/7(phaseVErr)
  [VMINDirVCurSenrCurErrNULL] -> Signal Conversion1/1
  Bus Selector/1 -> [VMINDirUCurSenrCurErrNULL]  "<VMIN_Dir_UCurSenrCurErr_NULL>"
  [VMINDirUCurSenrCurErrNULL] -> FaultState/6(phaseUErr)
  [VMINDirUCurSenrCurErrNULL] -> Signal Conversion/1
  Bus Selector/22 -> [VbMDSPDCBusCurValidflg]  "<VbMDSP_DCBusCurValid_flg>"
  [VbMDSPDCBusCurValidflg] -> DCBusCurrentValidDelay/1
  DCBus_Diagnostics/1(currentRaw) -> Bus Creator/41  "VfMDFM_DCBusCurrentRaw_A"
  DCBus_Diagnostics/2(currentSoft) -> Bus Creator/42  "VfMDFM_DCBusCurrentSoft_A"
  DCBus_Diagnostics/3(currentValid) -> Bus Creator/43  "VbMDFM_DCBusCurrentValid_flg"
  DCBus_Diagnostics/4(currentHardFault) -> DCBusCurrentHardFaultDelay/1, Bus Creator/44  "VbMDFM_DCBusCurrentHardFault_flg"
  DCBus_Diagnostics/5(currentSource) -> Bus Creator/45  "VuMDFM_DCBusCurrentSource_enum"
  DCBus_Diagnostics/6(voltageReport) -> Bus Creator/46  "VfMDFM_DCBusVoltReport_V"
  DCBusOperationalMin/1 -> DCBusOperationalAboveMin/2
  DCBusOperationalMax/1 -> DCBusOperationalBelowMax/2
  DCBusOperationalAboveMin/1 -> VoltageOperationalValid/1
  DCBusOperationalBelowMax/1 -> VoltageOperationalValid/2
  VoltageOperationalValid/1 -> Bus Creator/47  "VbMDFM_VoltageOperationalValid_flg"
  MDCC_outputs/1 -> Select_MDCC_DqSoftwareOverCurrent/1  "MDCC_output"
  Select_MDCC_DqSoftwareOverCurrent/1 -> DqSoftwareOverCurrent_Interface/1  "<VbMDCC_DqSoftwareOverCurrent_flg>"
  DqSoftwareOverCurrent_Interface/1 -> FaultState/10(dqSoftwareOverCurrent), Bus Creator/49  "VbMDFM_DqSoftwareOverCurrent_flg"
  [VMINDirUCurSenrCurErrNULL] -> PhaseSWOC_Qualifier/5(iuError)
  [VMINDirVCurSenrCurErrNULL] -> PhaseSWOC_Qualifier/6(ivError)
  [VMINDirWCurSenrCurErrNULL] -> PhaseSWOC_Qualifier/7(iwError)

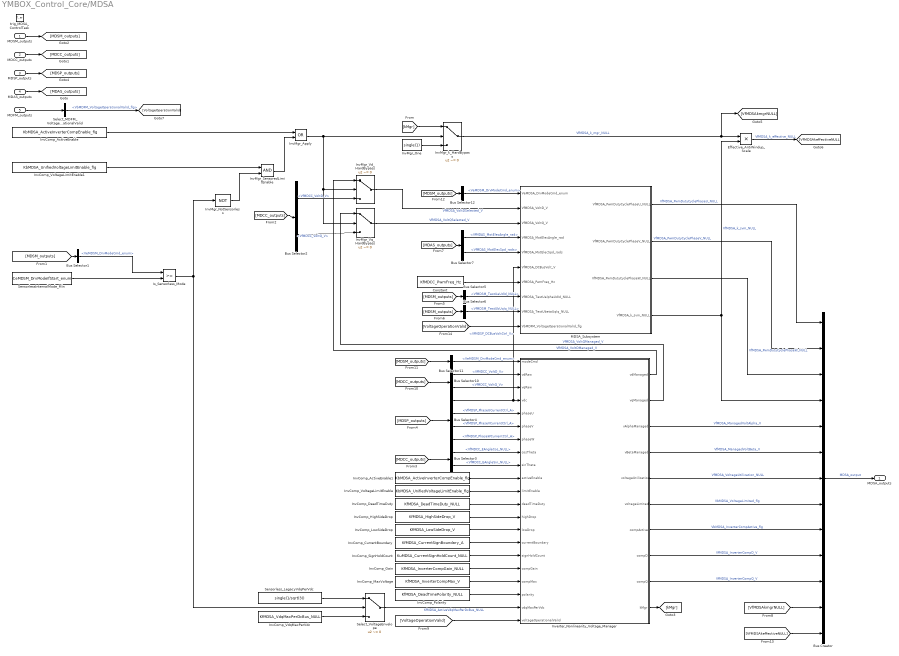
== system YMBOX_Control_Core/MDSA ==
  MDSM_outputs : Inport
  MDCC_outputs : Inport  Port=2
  MDSP_outputs : Inport  Port=3  OutDataTypeStr=Bus: MDSP_output
  MDAS_outputs : Inport  Port=4
  MDFM_outputs : Inport  Port=5  OutDataTypeStr=Bus: MDFM_output
  trig_MDSA_ControlTask : TriggerPort  TriggerType=function-call  VariantControl=(inherit)
  Bus Creator : BusCreator  Inputs=13  OutDataTypeStr=Bus: MDSA_output  NonVirtualBus=on
      settings: InheritFromInputs=off
  Bus Selector1 : BusSelector  OutputSignals=VeMDSM_DrvModeCmd_enum
  Bus Selector10 : BusSelector  OutputSignals=VfMDCC_VoltD_V,VfMDCC_VoltQ_V
  Bus Selector11 : BusSelector  OutputSignals=VeMDSM_DrvModeCmd_enum
  Bus Selector12 : BusSelector  OutputSignals=VeMDSM_DrvModeCmd_enum
  Bus Selector2 : BusSelector  OutputSignals=VfMDCC_VoltD_V,VfMDCC_VoltQ_V
  Bus Selector3 : BusSelector  OutputSignals=VfMDCC_EAngleCos_NULL,VfMDCC_EAngleSin_NULL
  Bus Selector4 : BusSelector  OutputSignals=VfMDSP_DCBusVoltCtrl_V,VfMDSP_PhaseUCurrentCtrl_A,VfMDSP_PhaseVCurrentCtrl_A,VfMDSP_PhaseWCurrentCtrl_A
  Bus Selector5 : BusSelector  OutputSignals=VfMDSM_TestUaUdId_NULL
  Bus Selector6 : BusSelector  OutputSignals=VfMDSM_TestUbUqIq_NULL
  Bus Selector7 : BusSelector  OutputSignals=VfMDAS_MotElecAngle_rad,VfMDAS_MotElecSpd_rads
  Constant : Constant  Value=KfMDCC_PwmFreq_Hz
  Effective_AntiWindup_Scale : Product  Inputs=**
  InvComp_ActiveEnable : Constant  Value=KbMDSA_ActiveInverterCompEnable_flg
  InvComp_ActiveEnable1 : Constant  Value=KbMDSA_ActiveInverterCompEnable_flg
  InvComp_CurrentBoundary : Constant  Value=KfMDSA_CurrentSignBoundary_A
  InvComp_DeadTimeDuty : Constant  Value=KfMDSA_DeadTimeDuty_NULL
  InvComp_Gain : Constant  Value=KfMDSA_InverterCompGain_NULL
  InvComp_HighSideDrop : Constant  Value=KfMDSA_HighSideDrop_V
  InvComp_LowSideDrop : Constant  Value=KfMDSA_LowSideDrop_V
  InvComp_MaxVoltage : Constant  Value=KfMDSA_InverterCompMax_V
  InvComp_Polarity : Constant  Value=KfMDSA_DeadTimePolarity_NULL
  InvComp_SignHoldCount : Constant  Value=KuMDSA_CurrentSignHoldCount_NULL
  InvComp_VdqMaxPerVdc : Constant  Value=KfMDSA_VdqMaxPerDcBus_NULL
  InvComp_VoltageLimitEnable : Constant  Value=KbMDSA_UnifiedVoltageLimitEnable_flg
  InvComp_VoltageLimitEnable1 : Constant  Value=KbMDSA_UnifiedVoltageLimitEnable_flg
  InvMgr_Apply : Logic  Operator=OR
  InvMgr_NotSensorless : Logic  Operator=NOT  Inputs=1
  InvMgr_One : Constant  Value=single(1)
  InvMgr_SensoredLimitEnable : Logic
  InvMgr_Vd_HardBypass : Switch  Criteria=u2 ~= 0
  InvMgr_Vq_HardBypass : Switch  Criteria=u2 ~= 0
  InvMgr_k_HardBypass : Switch  Criteria=u2 ~= 0
  Inverter_Nonlinearity_Voltage_Manager : Subsystem
  Is_Sensorless_Mode : RelationalOperator
  MDSA_Subsystem : Subsystem  TreatAsAtomicUnit=on  RTWFcnName=vPwm_MDSA  RTWFileName=MDSA
      settings: RTWSystemCode=Nonreusable function  RTWFcnNameOpts=User specified  RTWFileNameOpts=User specified
  Select_MDFM_VoltageOperationalValid : BusSelector  OutputSignals=VbMDFM_VoltageOperationalValid_flg
  Select_VoltageEnvelope : Switch  Criteria=u2 ~= 0
  SensorlessInternalMode_Min : Constant  Value=CeMDSM_DrvModeIfStart_enum
  Sensorless_LegacyVdqPerVdc : Constant  Value=single(1/sqrt(3))
  MDSA_outputs : Outport
  wires:
  MDSM_outputs/1 -> [MDSM_outputs]
  Inverter_Nonlinearity_Voltage_Manager/2(vqManaged) -> InvMgr_Vq_HardBypass/1  "VfMDSA_VoltQManaged_V"
  [MDSM_outputs] -> Bus Selector6/1
  MDAS_outputs/1 -> [MDAS_outputs]
  [MDSM_outputs] -> Bus Selector1/1
  Inverter_Nonlinearity_Voltage_Manager/7(compActive) -> Bus Creator/9  "VbMDSA_InverterCompActive_flg"
  SensorlessInternalMode_Min/1 -> Is_Sensorless_Mode/2
  Bus Selector2/1 -> InvMgr_Vd_HardBypass/3  "<VfMDCC_VoltD_V>"
  Bus Selector1/1 -> Is_Sensorless_Mode/1  "<VeMDSM_DrvModeCmd_enum>"
  [MDSM_outputs] -> Bus Selector5/1
  InvComp_DeadTimeDuty/1 -> Inverter_Nonlinearity_Voltage_Manager/12(deadTimeDuty)
  MDCC_outputs/1 -> [MDCC_outputs]
  InvComp_VdqMaxPerVdc/1 -> Select_VoltageEnvelope/3
  InvComp_VoltageLimitEnable/1 -> Inverter_Nonlinearity_Voltage_Manager/11(limitEnable)
  Bus Selector5/1 -> MDSA_Subsystem/8(VfMDSA_TestUalphaUdId_NULL)  "<VfMDSM_TestUaUdId_NULL>"
  Is_Sensorless_Mode/1 -> Select_VoltageEnvelope/2, InvMgr_NotSensorless/1
  Sensorless_LegacyVdqPerVdc/1 -> Select_VoltageEnvelope/1
  InvMgr_NotSensorless/1 -> InvMgr_SensoredLimitEnable/2
  [MDCC_outputs] -> Bus Selector2/1
  [MDAS_outputs] -> Bus Selector7/1
  Inverter_Nonlinearity_Voltage_Manager/8(compD) -> Bus Creator/10  "VfMDSA_InverterCompD_V"
  Select_VoltageEnvelope/1 -> Inverter_Nonlinearity_Voltage_Manager/20(vdqMaxPerVdc)  "KfMDSA_ActiveVdqMaxPerDcBus_NULL"
  InvMgr_SensoredLimitEnable/1 -> InvMgr_Apply/2
  InvMgr_Vq_HardBypass/1 -> MDSA_Subsystem/3(VfMDSA_VoltQ_V)  "VfMDSA_VoltQSelected_V"
  Bus Selector2/2 -> InvMgr_Vq_HardBypass/3  "<VfMDCC_VoltQ_V>"
  InvComp_Polarity/1 -> Inverter_Nonlinearity_Voltage_Manager/19(polarity)
  InvComp_SignHoldCount/1 -> Inverter_Nonlinearity_Voltage_Manager/16(signHoldCount)
  Bus Selector7/1 -> MDSA_Subsystem/4(VfMDSA_MotElecAngle_rad)  "<VfMDAS_MotElecAngle_rad>"
  Bus Selector7/2 -> MDSA_Subsystem/5(VfMDSA_MotElecSpd_rads)  "<VfMDAS_MotElecSpd_rads>"
  Bus Selector6/1 -> MDSA_Subsystem/9(VfMDSA_TestUbetaUqIq_NULL)  "<VfMDSM_TestUbUqIq_NULL>"
  InvComp_HighSideDrop/1 -> Inverter_Nonlinearity_Voltage_Manager/13(highDrop)
  InvComp_LowSideDrop/1 -> Inverter_Nonlinearity_Voltage_Manager/14(lowDrop)
  InvComp_CurrentBoundary/1 -> Inverter_Nonlinearity_Voltage_Manager/15(currentBoundary)
  MDSA_Subsystem/4(VfMDSA_k_svm_NULL) -> Effective_AntiWindup_Scale/2, Bus Creator/4  "VfMDSA_k_svm_NULL"
  InvComp_Gain/1 -> Inverter_Nonlinearity_Voltage_Manager/17(compGain)
  InvComp_MaxVoltage/1 -> Inverter_Nonlinearity_Voltage_Manager/18(compMax)
  InvMgr_Apply/1 -> InvMgr_Vd_HardBypass/2, InvMgr_Vq_HardBypass/2, InvMgr_k_HardBypass/2
  Inverter_Nonlinearity_Voltage_Manager/4(vBetaManaged) -> Bus Creator/6  "VfMDSA_ManagedVoltBeta_V"
  Inverter_Nonlinearity_Voltage_Manager/1(vdManaged) -> InvMgr_Vd_HardBypass/1  "VfMDSA_VoltDManaged_V"
  Inverter_Nonlinearity_Voltage_Manager/3(vAlphaManaged) -> Bus Creator/5  "VfMDSA_ManagedVoltAlpha_V"
  Inverter_Nonlinearity_Voltage_Manager/5(voltageUtilization) -> Bus Creator/7  "VfMDSA_VoltageUtilization_NULL"
  Inverter_Nonlinearity_Voltage_Manager/6(voltageLimited) -> Bus Creator/8  "VbMDSA_VoltageLimited_flg"
  Inverter_Nonlinearity_Voltage_Manager/9(compQ) -> Bus Creator/11  "VfMDSA_InverterCompQ_V"
  InvMgr_Vd_HardBypass/1 -> MDSA_Subsystem/2(VfMDSA_VoltD_V)  "VfMDSA_VoltDSelected_V"
  Constant/1 -> MDSA_Subsystem/7(VfMDSA_PwmFreq_Hz)
  MDSA_Subsystem/3(VfMDSA_PwmDutyCyclePhaseW_NULL) -> Bus Creator/3  "VfMDSA_PwmDutyCyclePhaseW_NULL"
  MDSA_Subsystem/2(VfMDSA_PwmDutyCyclePhaseV_NULL) -> Bus Creator/2  "VfMDSA_PwmDutyCyclePhaseV_NULL"
  MDSA_Subsystem/1(VfMDSA_PwmDutyCyclePhaseU_NULL) -> Bus Creator/1  "VfMDSA_PwmDutyCyclePhaseU_NULL"
  Bus Creator/1 -> MDSA_outputs/1  "MDSA_output"
  [MDCC_outputs] -> Bus Selector3/1
  InvComp_ActiveEnable1/1 -> Inverter_Nonlinearity_Voltage_Manager/10(activeEnable)
  [MDSP_outputs] -> Bus Selector4/1
  Bus Selector4/1 -> MDSA_Subsystem/6(VfMDSA_DCBusVolt_V), Inverter_Nonlinearity_Voltage_Manager/4(vdc)  "<VfMDSP_DCBusVoltCtrl_V>"
  [MDCC_outputs] -> Bus Selector10/1
  Bus Selector10/1 -> Inverter_Nonlinearity_Voltage_Manager/2(vdRaw)  "<VfMDCC_VoltD_V>"
  Bus Selector10/2 -> Inverter_Nonlinearity_Voltage_Manager/3(vqRaw)  "<VfMDCC_VoltQ_V>"
  [MDSM_outputs] -> Bus Selector11/1
  Bus Selector11/1 -> Inverter_Nonlinearity_Voltage_Manager/1(modeCmd)  "<VeMDSM_DrvModeCmd_enum>"
  [MDSM_outputs] -> Bus Selector12/1
  Bus Selector12/1 -> MDSA_Subsystem/1(VeMDSA_DrvModeCmd_enum)  "<VeMDSM_DrvModeCmd_enum>"
  InvComp_ActiveEnable/1 -> InvMgr_Apply/1
  InvComp_VoltageLimitEnable1/1 -> InvMgr_SensoredLimitEnable/1
  InvMgr_One/1 -> InvMgr_k_HardBypass/3
  InvMgr_k_HardBypass/1 -> [VfMDSAkmgrNULL], Effective_AntiWindup_Scale/1  "VfMDSA_k_mgr_NULL"
  Inverter_Nonlinearity_Voltage_Manager/10(kMgr) -> [kMgr]
  [kMgr] -> InvMgr_k_HardBypass/1
  [VfMDSAkmgrNULL] -> Bus Creator/12
  Effective_AntiWindup_Scale/1 -> [VfMDSAkeffectiveNULL]  "VfMDSA_k_effective_NULL"
  [VfMDSAkeffectiveNULL] -> Bus Creator/13
  Bus Selector3/1 -> Inverter_Nonlinearity_Voltage_Manager/8(cosTheta)  "<VfMDCC_EAngleCos_NULL>"
  Bus Selector3/2 -> Inverter_Nonlinearity_Voltage_Manager/9(sinTheta)  "<VfMDCC_EAngleSin_NULL>"
  Bus Selector4/2 -> Inverter_Nonlinearity_Voltage_Manager/5(phaseU)  "<VfMDSP_PhaseUCurrentCtrl_A>"
  Bus Selector4/3 -> Inverter_Nonlinearity_Voltage_Manager/6(phaseV)  "<VfMDSP_PhaseVCurrentCtrl_A>"
  Bus Selector4/4 -> Inverter_Nonlinearity_Voltage_Manager/7(phaseW)  "<VfMDSP_PhaseWCurrentCtrl_A>"
  MDSP_outputs/1 -> [MDSP_outputs]
  MDFM_outputs/1 -> Select_MDFM_VoltageOperationalValid/1
  [VoltageOperationValid] -> Inverter_Nonlinearity_Voltage_Manager/21(voltageOperationalValid)
  [VoltageOperationValid] -> MDSA_Subsystem/10(VbMDFM_VoltageOperationalValid_flg)
  Select_MDFM_VoltageOperationalValid/1 -> [VoltageOperationValid]  "<VbMDFM_VoltageOperationalValid_flg>"

== system YMBOX_Control_Core/MDSM ==
  MDSP_outputs : Inport
  MDAS_outputs : Inport  Port=2
  MDFM_outputs : Inport  Port=3
  trig_MDSM_ControlTask : TriggerPort  TriggerType=function-call  VariantControl=(inherit)
  Bus Creator : BusCreator  Inputs=9
  Bus Selector : BusSelector  OutputSignals=Direct_Output.VMIN_Dir_TestUaUdId_NULL,Direct_Output.VMIN_Dir_TestUbUqIq_NULL,Direct_Output.VMIN_ECAN_MotTrgtTq_Nm,Direct_Output.VMIN_ECAN_MotTrgtSpd_rpm,Direct_Output.VMIN_ECAN_MotWrkMd_enum,Direct_Output.VMIN_ECAN_MCUEnb_flg
  Cast_MDAS_SmoReady_uint8 : DataTypeConversion  OutDataTypeStr=uint8  SaturateOnIntegerOverflow=off  RndMeth=Floor
  Dly_MDAS_SmoReady : UnitDelay  InitialCondition=false  SampleTime=-1  HasFrameUpgradeWarning=on
  Expose_DrvModeReq_uint16 : DataTypeConversion  OutDataTypeStr=uint16  SaturateOnIntegerOverflow=off  RndMeth=Floor
  FaultGated_Enable : Logic  AllPortsSameDT=off  OutDataTypeStr=boolean
  FaultStop_Not : Logic  Operator=NOT  Inputs=1  AllPortsSameDT=off  OutDataTypeStr=boolean
  MDSM_ModeManager : Subsystem
      settings: AttributesFormatString=|
      | VARIANT ROUTE + GENERIC SUPERVISOR
      | compile mode = external mode 6 / 7 / 8 / 9 / 10
      | runtime: STAGE1 -> optional STAGE2
  Select_MDAS_ObserverReady : BusSelector  OutputSignals=VbMDAS_SmoReady_flg
  Select_MDFM_StopRequest : BusSelector  OutputSignals=VbMDFM_StopRequest_flg
  Signal Conversion{,1..3} (4 alike) : SignalConversion  OverrideOpt=off
  Write_MDTM_Reset : DataStoreWrite  DataStoreName=MDTM_ResetDispatch  IndexOptions=Index vector (dialog)  Indices=1  OutputSizes=1
  MDSM_outputs : Outport
  wires:
  Cast_MDAS_SmoReady_uint8/1 -> MDSM_ModeManager/3(VbMDAS_SmoReady_flg)
  MDAS_outputs/1 -> Select_MDAS_ObserverReady/1
  Bus Creator/1 -> MDSM_outputs/1  "MDSM_output"
  Bus Selector/4 -> MDSM_ModeManager/4(VfMDSM_TrgtSpd_rpm), Signal Conversion3/1  "<VMIN_ECAN_MotTrgtSpd_rpm>"
  Bus Selector/3 -> Signal Conversion2/1  "<VMIN_ECAN_MotTrgtTq_Nm>"
  Bus Selector/2 -> Signal Conversion1/1  "<VMIN_Dir_TestUbUqIq_NULL>"
  Bus Selector/1 -> Signal Conversion/1  "<VMIN_Dir_TestUaUdId_NULL>"
  Bus Selector/5 -> MDSM_ModeManager/1(VeMDSM_DrvModeReq_enum), Expose_DrvModeReq_uint16/1  "<VMIN_ECAN_MotWrkMd_enum>"
  MDSP_outputs/1 -> Bus Selector/1
  Dly_MDAS_SmoReady/1 -> Cast_MDAS_SmoReady_uint8/1
  MDSM_ModeManager/1(VeMDSM_DrvModeCmd_enum) -> Bus Creator/1  "VeMDSM_DrvModeCmd_enum"
  MDSM_ModeManager/2(VbMDTM_PiReset_flg) -> Write_MDTM_Reset/1, Bus Creator/2  "VbMDTM_PiReset_flg"
  MDSM_ModeManager/3(VbMDCC_PiReset_flg) -> Bus Creator/3  "VbMDCC_PiReset_flg"
  MDSM_ModeManager/4(VuMDFM_FFEnable_enum) -> Bus Creator/4  "VeMDFM_FFEnable_enum"
  Signal Conversion/1 -> Bus Creator/5  "VfMDSM_TestUaUdId_NULL"
  Signal Conversion1/1 -> Bus Creator/6  "VfMDSM_TestUbUqIq_NULL"
  Signal Conversion2/1 -> Bus Creator/7  "VfMDSM_TrgtTq_Nm"
  Signal Conversion3/1 -> Bus Creator/8  "VfMDSM_TrgtSpd_rpm"
  Expose_DrvModeReq_uint16/1 -> Bus Creator/9  "VeMDSM_DrvModeReq_enum"
  Select_MDAS_ObserverReady/1 -> Dly_MDAS_SmoReady/1  "<VbMDAS_SmoReady_flg>"
  MDFM_outputs/1 -> Select_MDFM_StopRequest/1
  Select_MDFM_StopRequest/1 -> FaultStop_Not/1  "<VbMDFM_StopRequest_flg>"
  Bus Selector/6 -> FaultGated_Enable/1  "<VMIN_ECAN_MCUEnb_flg>"
  FaultStop_Not/1 -> FaultGated_Enable/2
  FaultGated_Enable/1 -> MDSM_ModeManager/2(VbMDSM_MCUEnb_flg)
